simulink model "SMXQ6_600_GoKart_Project"  (R2026a)
settings: Solver=VariableStepAuto  StopTime=7
model workspace (MAT data in the model file):
  CruiseSpeed = 1
  DaxisKi = 3000
  DaxisKp = 18
  InvThresh = 1
  MaxPower = 2638
  MaxTorque = 42
  NPP = 20
  QaxisKi = 3000
  QaxisKp = 18
  SpeedKi = 2882.18001217
  SpeedKp = 90.4773949421
  Tf = 0.0001
  Ts = 0.0001
  Vdc = 320
  flux = 0.103309826163
  speedramp = [0 0.125 0.125 0.5 0.5 1 1]
  timeramp = [0 1 2 3 4 5 6]
libraries: fl_lib x15, nesl_utility x15, sdl_lib x6, ee_lib x4, slpidlib x1, eePmsmFieldOrientedControl x1
(part 1 of 2)
settings Model: Creator=bneiswan  LastModifiedBy=Uriel
settings SimscapeCC: SimscapeNominalValues="[{\"value\":\"1\",\"unit\":\"A\"},{\"value\":\"1\",\"unit\":\"bar\"},{\"value\":\"1\",\"unit\":\"cm^2\"},{\"value\":\"1\",\"unit\":\"cm^3/s\"},{\"value\":\"1\",\"unit\":\"kJ/kg\"},{\"value\":\"1\",\"unit\":\"kW\"},{\"value\":\"1\",\"unit\":\"l\"},{\"value\":\"1\",\"unit\":\"N\"},{\"value\":\"1\",\"unit\":\"N*m\"},{\"value\":\"1\",\"unit\":\"V\"}]"  SimscapeLogType=none  SimscapeLogDataHistory=5000.0

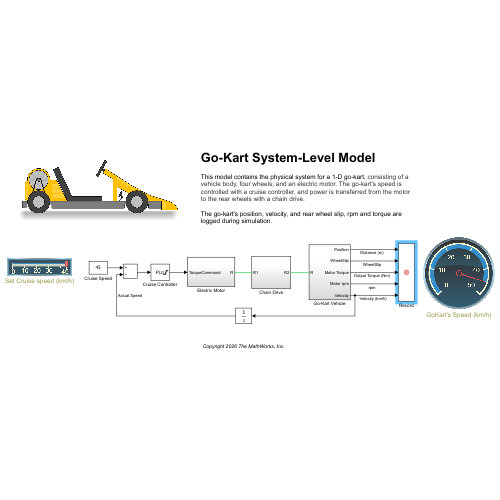
[thumbnail: Simulink's stored preview of the top-level diagram]
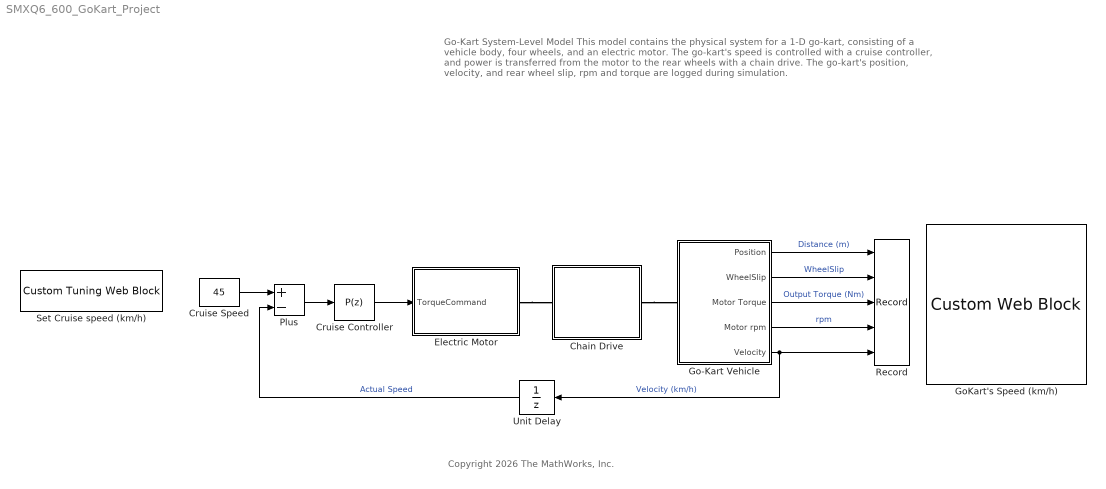
== system SMXQ6_600_GoKart_Project ==
  note: Copyright 2026 The MathWorks, Inc.
  note: Go-Kart System-Level Model
      |
      | This model contains the physical system for a 1-D go-kart, consisting of a vehicle body, four wheels, and an electric motor. The go-kart's speed is controlled with a cruise controller, and power is transferred from the motor to the rear wheels with a chain drive.
      |
      | The go-kart's position, velocity, and rear wheel slip, rpm and torque are logged during simulation.
  Chain Drive : Subsystem
  Cruise Controller : slpidlib/PID Controller  Controller=P  Form=Parallel  TimeDomain=Discrete-time  UseExternalTs=off  SampleTime=-1  IntegratorMethod=Forward Euler  FilterMethod=Forward Euler  ControllerParametersSource=internal  P=250  I=.25  UseKiTs=off  D=10  UseExternalDerivativeSource=off  N=100  UseFilter=on  TunerSelectOption=Transfer Function Based (PID Tuner App)  InitialConditionSource=internal  InitialConditionForIntegrator=0  InitialConditionForFilter=0  DifferentiatorICPrevScaledInput=0  ExternalReset=none  TrackingMode=off  Kt=1  LimitOutput=on  SatLimitsSource=internal  UpperSaturationLimit=42  LowerSaturationLimit=0  LinearizeAsGain=on  AntiWindupMode=none  Kb=1  LimitIntegrator=off  UpperIntegratorSaturationLimit=inf  LowerIntegratorSaturationLimit=-inf  POutMin=[]  POutMax=[]  IOutMin=[]  IOutMax=[]  DOutMin=[]  DOutMax=[]  NOutMin=[]  NOutMax=[]  SumOutMin=[]  SumOutMax=[]  SaturationOutMin=[]  SaturationOutMax=[]  PParamMin=[]  PParamMax=[]  IParamMin=[]  IParamMax=[]  DParamMin=[]  DParamMax=[]  NParamMin=[]  NParamMax=[]  KbParamMin=[]  KbParamMax=[]  KtParamMin=[]  KtParamMax=[]  KbOutMin=[]  KbOutMax=[]  KtOutMin=[]  KtOutMax=[]  IntegratorOutMin=[]  IntegratorOutMax=[]  FilterOutMin=[]  FilterOutMax=[]  SumI1OutMin=[]  SumI1OutMax=[]  SumI2OutMin=[]  SumI2OutMax=[]  SumI3OutMin=[]  SumI3OutMax=[]  SumI4OutMin=[]  SumI4OutMax=[]  SumDOutMin=[]  SumDOutMax=[]  DifferentiatorOutMin=[]  DifferentiatorOutMax=[]  FilterDiffOutCoefMin=[]  FilterDiffOutCoefMax=[]  ReciprocalOutMin=[]  ReciprocalOutMax=[]  SumDenOutMin=[]  SumDenOutMax=[]  SumNumOutMin=[]  SumNumOutMax=[]  DivideOutMin=[]  DivideOutMax=[]  UdiffTsProdOutMin=[]  UdiffTsProdOutMax=[]  NTsProdOutMin=[]  NTsProdOutMax=[]  UintegralTsProdOutMin=[]  UintegralTsProdOutMax=[]  UngainTsProdOutMin=[]  UngainTsProdOutMax=[]  ClampingZeroOutDataTypeStr=Inherit: Inherit via back propagation  ClampingZeroOutMin=[]  ClampingZeroOutMax=[]  FilterDenConstantOutDataTypeStr=Inherit: Inherit via back propagation  FilterDenConstantOutMin=[]  FilterDenConstantOutMax=[]  PCopyOutDataTypeStr=Inherit: Inherit via back propagation  PCopyOutMin=[]  PCopyOutMax=[]  NCopyOutDataTypeStr=Inherit: Inherit via back propagation  NCopyOutMin=[]  NCopyOutMax=[]  IntegratorContinuousStateAttributes=''  IntegratorStateMustResolveToSignalObject=off  IntegratorRTWStateStorageClass=Auto  FilterContinuousStateAttributes=''  FilterStateMustResolveToSignalObject=off  FilterRTWStateStorageClass=Auto  ParallelPVariant=InternalParameters  IdealPVariant=Disabled  IVariant=Disabled  DVariant=Disabled  IntegratorVariant=Disabled  SatVariant=Enabled  AWVariant=Disabled  PCopyVariant=Disabled  TRVariant=Disabled  FdbkBlocksVariant=Forward  IdealPFdbkVariant=Disabled  SatFdbkVariant=Disabled  DerivativeFilterVariant=Disabled  NVariant=Disabled  NCopyVariant=Disabled_SignalSpec  FilterICVariant=Disabled  IntegratorICVariant=Disabled  ExternalResetVariant=Disabled  TRSumVariant=Passthrough  SumFdbkVariant=Disabled  SumVariant=Passthrough_P  TsampFilterVariant=InternalTs  TsampNgainVariant=Passthrough  TsampIntegralVariant=Disabled_SignalSpec  ExternalSaturationOutDataTypeStr=Inherit: Same as second input  DerivativeSourceVariant=Disabled  PreIntVariant=InternalPreInt
  Cruise Speed : Constant  Value=45
  Electric Motor : Subsystem
      settings: PortSchema="{\"entries\":[{\"content\":{\"sides\":[{\"content\":{\"connectorIds\":[\"LConn1\"]},\"type\":\"ConnectorPlacement.EquallySpacedRectSide\",\"uuid\":\"f2a7d976-2b6b-46c6-a0c1-1e92cd96bdba\"},{\"content\":{\"connectorIds\":[\"In1\"],\"side\":\"RIGHT\"},\"type\":\"ConnectorPlacement.EquallySpacedRectSide\",\"uuid\":\"0fb82cfe-b0ae-4149-8652-d7e7f0635458\"},{\"content\":{\"side\":\"TOP\"},\"type\":\"ConnectorPlacement.EquallySpacedRectSide\",\"uuid\":\"f6564529-e6f3-4994-b1c4-046997b74a0b\"}]},\"type\":\"ConnectorPlacement.EquallySpacedConnector\",\"uuid\":\"916fedef-c12c-4718-8891-25d762e09ffe\"}],\"packageUris\":[\"http://schema.mathworks.com/mf0/Connector/R2020b\"],\"version\":\"1.0\"}"
  Go-Kart Vehicle : Subsystem
  GoKart's Speed (km/h) : CustomWebBlock  LabelPosition=Hide  ShowInitialText=on  Configuration="{\"components\":[{\"name\":\"CircularScaleComponent\",\"settings\":{\"bounds\":{\"max\":50,\"min\":0,\"tickInterval\":5},\"direction\":\"cw\",\"flipLimits\":0,\"innerRadius\":0.75,\"internalTickHeightScaleFactor\":1,\"labelColor\":[255,255,200],\"labelFont\":{\"font\":\"Arial\",\"fontSize\":12},\"labelRadius\":0.528,\"labelTransparency\":1,\"minorTickHeightScaleFactor\":0.2,\"needleImage\":{\"size\":[200,50],\"src\":\"data:image\\/svg+xml;base64,PD94bWwgdmVyc2lvbj0iMS4wIiBlbmNvZGluZz0idXRmLTgiPz4KPCEtLSBHZW5lcmF0b3I6IEFkb2JlIElsbHVzdHJhdG9yIDI0LjEuMiwgU1ZHIEV4cG9ydCBQbHVnLUluIC4gU1ZHIFZlcnNpb246IDYuMDAgQnVpbGQgMCkgIC0tPgo8c3ZnIHZlcnNpb249IjEuMSIgaWQ9IkxheWVyXzEiIHhtbG5zPSJodHRwOi8vd3d3LnczLm9yZy8yMDAwL3N2ZyIgeG1sbnM6eGxpbms9Imh0dHA6Ly93d3cudzMub3JnLzE5OTkveGxpbmsiIHg9IjBweCIgeT0iMHB4IgoJIHZpZXdCb3g9IjAgMCAyMDAgNTAiIHN0eWxlPSJlbmFibGUtYmFja2dyb3VuZDpuZXcgMCAwIDIwMCA1MDsiIHhtbDpzcGFjZT0icHJlc2VydmUiPgo8c3R5bGUgdHlwZT0idGV4dC9jc3MiPgoJLnN0MHtmaWxsOiNFQzIxMjc7fQo8L3N0eWxlPgo8cGF0aCBjbGFzcz0ic3QwIiBkPSJNMTYyLjgsMTMuN0MxNjksNC40LDE4MS43LDEuOSwxOTEsOC4xczExLjgsMTguOSw1LjYsMjguMnMtMTguOSwxMS44LTI4LjIsNS42bDAsMAoJQzE1OS4xLDM1LjYsMTU2LjYsMjMsMTYyLjgsMTMuN0wxNjIuOCwxMy43eiBNMTY1LjgsMTUuOGMtNS4xLDcuNi0zLjEsMTcuOSw0LjYsMjNjNy42LDUuMSwxNy45LDMuMSwyMy00LjYKCWM1LjEtNy42LDMuMS0xNy45LTQuNi0yM2wwLDBDMTgxLjIsNi4yLDE3MC45LDguMiwxNjUuOCwxNS44eiIvPgo8cGF0aCBjbGFzcz0ic3QwIiBkPSJNMC40LDI1Ljl2LTMuM2wxNTktMi41Yy0wLjcsMi42LTAuNyw1LjIsMCw3LjhMMC40LDI1Ljl6Ii8+CjxjaXJjbGUgY2xhc3M9InN0MCIgY3g9IjE3OS42IiBjeT0iMjQiIHI9IjAuNyIvPgo8L3N2Zz4K\"},\"needleOffset\":[0.18464878250906522,0],\"needleOrientation\":-45,\"needleRotation\":180,\"needleSize\":{\"height\":0.11741692305346914,\"width\":0.46108337545091255},\"outerRadius\":0.9,\"position\":[0.05,0.05,0.9,0.9],\"referencePoint\":\"auto\",\"scaleAngle\":270,\"scaleAngleOffset\":135,\"scaleColors\":[],\"scaleColorsSize\":0.2,\"scaleDirection\":\"CW\",\"scalePosition\":[0,0,1,1],\"showLabels\":1,\"showMinorTicks\":1,\"showSpanLine\":1,\"showTicks\":1,\"tickColor\":[252,252,197],\"tickTransparency\":1,\"valueBarColor\":[0,114,189],\"valueBarPosition\":[0,0,1,1],\"valueBarSize\":0.2,\"valueBarTransparency\":1}},{\"name\":\"BackgroundImageComponent\",\"settings\":{\"image\":{\"size\":[500,500],\"src\":\"data:image\\/svg+xml;base64,PD94bWwgdmVyc2lvbj0iMS4wIiBlbmNvZGluZz0iVVRGLTgiIHN0YW5kYWxvbmU9Im5vIj8+CjxzdmcKICAgeG1sbnM6ZGM9Imh0dHA6Ly9wdXJsLm9yZy9kYy9lbGVtZW50cy8xLjEvIgogICB4bWxuczpjYz0iaHR0cDovL2NyZWF0aXZlY29tbW9ucy5vcmcvbnMjIgogICB4bWxuczpyZGY9Imh0dHA6Ly93d3cudzMub3JnLzE5OTkvMDIvMjItcmRmLXN5bnRheC1ucyMiCiAgIHhtbG5zOnN2Zz0iaHR0cDovL3d3dy53My5vcmcvMjAwMC9zdmciCiAgIHhtbG5zPSJodHRwOi8vd3d3LnczLm9yZy8yMDAwL3N2ZyIKICAgeG1sbnM6 ...(+9964 chars)\"},\"position\":[0,0,1,1],\"scaleMode\":\"0\"}},{\"name\":\"ForegroundImageComponent\",\"settings\":{\"image\":{\"size\":[0,0],\"src\":\"default\",\"srcOrientation\":[]},\"isForeground\":1,\"position\":[0,0,1,1],\"scaleMode\":\"0\"}}],\"derived\":{\"blockParameters\":{\"ForegroundColor\":[0.9882352941176471,0.9882352941176471,0.7725490196078432],\"Limits\":{\"Max\":50,\"Min\":0,\"Ticks\":5},\"ScaleColors\":[],\"ScaleDirection\":\"Clockwise\",\"ScaleMax\":50,\"ScaleMin\":0,\"TickInterval\":5,\"fixedAspectRatio\":\"on\"}},\"settings\":{\"BindingType\":\"signal\",\"aspectRatio\":1.032258064516129,\"backgroundColor\":[0,0,0,\"1\"],\"backgroundOffset\":1,\"backgroundOpacity\":1,\"direction\":\"cw\",\"fixedAspectRatio\":\"on\",\"flipLimits\":0,\"orientation\":\"horizontal\",\"showBackgroundColor\":false,\"value\":0,\"version\":\"R2023a\"},\"type\":\"CircularGauge\"}"
  Plus : Sum  Inputs=+-
  Record : Record  NumPorts=5.0  FileSettingsInternal="{\"entries\":[{\"content\":{\"excelSettings\":{\"content\":{},\"type\":\"Streamout.ExcelSettings\"},\"parquetSettings\":{\"content\":{},\"type\":\"Streamout.ParquetSettings\"}},\"type\":\"Streamout.FileSettingStorage\",\"uuid\":\"\"}],\"packageUris\":[\"http:\\/\\/schema.mathworks.com\\/mf0\\/streamout_blocks\\/R2020a\"],\"version\":\"1.0\"}"  FrameSettings=[0, 0, 0, 0, 0]  SignalsInternal="{\"entries\":[{\"content\":{\"signals\":[{\"content\":{\"blockPath\":[],\"dimensions\":[1],\"domain\":\"\",\"lineColor\":\"#0072bd\",\"lineWidth\":2,\"plots\":[ 1 ],\"port\":1,\"sid\":[\"\"],\"signalID\":1,\"signalName\":\"Distance (m)\"},\"type\":\"RecordBlkView.Signal\",\"uuid\":\"\"},{\"content\":{\"blockPath\":[],\"dimensions\":[1],\"domain\":\"\",\"lineColor\":\"#d95319\",\"lineWidth\":2,\"plots\":[ 1 ],\"port\":2,\"sid\":[\"\"],\"signalID\":2,\"signalName\":\"WheelSlip\"},\"type\":\"RecordBlkView.Signal\",\"uuid\":\"\"},{\"content\":{\"blockPath\":[],\"dimensions\":[1],\"domain\":\"\",\"lineColor\":\"#edb120\",\"lineWidth\":2,\"plots\":[ 1 ],\"port\":3,\"sid\":[\"\"],\"signalID\":3,\"signalName\":\"Output Torque (Nm)\"},\"type\":\"RecordBlkView.Signal\",\"uuid\":\"\"},{\"content\":{\"blockPath\":[],\"dimensions\":[1],\"domain\":\"\",\"lineColor\":\"#7e2f8e\",\"lineWidth\":2,\"plots\":[ 1 ],\"port\":4,\"sid\":[\"\"],\"signalID\":4,\"signalName\":\"rpm\"},\"type\":\"RecordBlkView.Signal\",\"uuid\":\"\"},{\"content\":{\"blockPath\":[],\"dimensions\":[1],\"domain\":\"\",\"lineColor\":\"#77ac30\",\"lineWidth\":2,\"plots\":[ 1 ],\"port\":5,\"sid\":[\"\"],\"signalID\":5,\"signalName\":\"Velocity (km\\/h)\"},\"type\":\"RecordBlkView.Signal\",\"uuid\":\"\"}]},\"type\":\"RecordBlkView.InputSignals\",\"uuid\":\"\"}],\"packageUris\":[\"http:\\/\\/schema.mathworks.com\\/mf0\\/streamout_blocks\\/R2020a\"],\"version\":\"1.0\"}"  VisualizationBindings="{\"sparklinesplugin\":{\"info\":[{\"bindingParametersList\":[],\"subplotID\":1}]}}"
  Set Cruise speed (km/h) : CustomTuningWebBlock  LabelPosition=Hide  ShowInitialText=on  Configuration="{\"components\":[{\"name\":\"LinearScaleComponent\",\"settings\":{\"bounds\":{\"max\":45,\"min\":0,\"tickInterval\":\"auto\"},\"internalTickHeightScaleFactor\":0.5,\"labelColor\":[255,255,200],\"labelFont\":{\"font\":\"Arial\",\"fontSize\":12},\"labelOffset\":0.05,\"labelTransparency\":1,\"needleImage\":{\"size\":[596,842],\"src\":\"data:image\\/svg+xml;base64,PD94bWwgdmVyc2lvbj0iMS4wIiBlbmNvZGluZz0idXRmLTgiPz4NCjwhLS0gR2VuZXJhdG9yOiBBZG9iZSBJbGx1c3RyYXRvciAyNS4wLjAsIFNWRyBFeHBvcnQgUGx1Zy1JbiAuIFNWRyBWZXJzaW9uOiA2LjAwIEJ1aWxkIDApICAtLT4NCjxzdmcgdmVyc2lvbj0iMS4xIg0KCSBpZD0ic3ZnOCIgeG1sbnM6Y2M9Imh0dHA6Ly9jcmVhdGl2ZWNvbW1vbnMub3JnL25zIyIgeG1sbnM6ZGM9Imh0dHA6Ly9wdXJsLm9yZy9kYy9lbGVtZW50cy8xLjEvIiB4bWxuczppbmtzY2FwZT0iaHR0cDovL3d3dy5pbmtzY2FwZS5vcmcvbmFtZXNw ...(+2420 chars)\",\"srcOrientation\":\"Right\"},\"needleOffset\":[-0.8044596912521441,-0.0642123287671233],\"needleSize\":{\"height\":0.4337797619047619,\"width\":0.07668067226890757},\"position\":[0.2829861111111111,0.04398634453781513,0.9196428571428571,0.6088789682539683],\"referencePoint\":\"auto\",\"scaleColors\":[],\"scaleColorsSize\":0.2,\"scaleDirection\":\"LR\",\"showLabels\":1,\"showMinorTicks\":0,\"showSpanLine\":1,\"showTicks\":1,\"tickColor\":[252,252,197],\"tickTransparency\":1,\"valueBarColor\":[0,114,189],\"valueBarOffset\":-0.27,\"valueBarSize\":0.1,\"valueBarTransparency\":1}},{\"name\":\"BackgroundImageComponent\",\"settings\":{\"image\":{\"size\":[380,101],\"src\":\"data:image\\/svg+xml;base64,PHN2ZyB4bWxucz0iaHR0cDovL3d3dy53My5vcmcvMjAwMC9zdmciIHhtbG5zOnhsaW5rPSJodHRwOi8vd3d3LnczLm9yZy8xOTk5L3hsaW5rIiB2aWV3Qm94PSIwIDAgMzgwIDEwMSI+PGRlZnM+PHN0eWxlPi5jbHMtMXtmaWxsOiMwMDJiNDI7fS5jbHMtMntmaWxsOiM0MjcwODI7fS5jbHMtM3tmaWxsOnVybCgjcmFkaWFsLWdyYWRpZW50KTt9LmNscy00e2ZpbGw6I2M4YzhjODtzdHJva2U6IzAwMDt9PC9zdHlsZT48cmFkaWFsR3JhZGllbnQgaWQ9InJhZGlhbC1ncmFkaWVudCIgY3g9IjE5MCIgY3k9IjUwLjUiIHI9IjI2OS4yMSIgZ3JhZGllbnRVbml0cz0idXNlclNwYWNlT25Vc2UiPjxzdG9wIG9mZnNldD0iMC4wMSIgc3RvcC1jb2xvcj0iIzNlNGY1OCIvPjxzdG9wIG9mZnNldD0iMC4wNiIgc3RvcC1jb2xvcj0iIzQ0NTc2MSIvPjxzdG9wIG9mZnNldD0iMC4xNSIgc3RvcC1jb2xvcj0iIzU1NmE3NiIvPjxzdG9wIG9mZnNldD0iMC4yNSIgc3RvcC1jb2xvcj0iIzZkODg5NSIvPjxzdG9wIG9mZnNldD0iMC4zOCIgc3RvcC1jb2xvcj0iIzhmYjJjMyIvPjxzdG9wIG9mZnNldD0iMC41MiIgc3RvcC1jb2xvcj0iI2I2ZTRmYSIvPjxzdG9wIG9mZnNldD0iMSIgc3RvcC1jb2xvcj0iIzE1NDY1NyIvPjwvcmFkaWFsR3JhZGllbnQ+PC9kZWZzPjxnIGlkPSJmcmFtZSI+PGcgaWQ9IkxheWVyXzIiIGRhdGEtbmFtZT0iTGF5ZXIgMiI+PGcgaWQ9IkxheWVyXzEtMiIgZGF0YS1uYW1lPSJMYXllciAxLTIiPjxyZWN0IGlkPSJyZWN0MTAzNiIgY2xhc3M9ImNscy0xIiB4PSIxMSIgeT0iMTEiIHdpZHRoPSIzNTgiIGhlaWdodD0iNzkiLz48cGF0aCBpZD0icGF0aDEwMzgiIGNsYXNzPSJjbHMtMiIgZD0iTTgsOFY5M0gzNzJWOFpNMzY5LDkwSDExVjExSDM2OVoiLz48cGF0aCBpZD0icGF0aDEwNDAiIGNsYXNzPSJjbHMtMyIgZD0iTTAsMFYxMDFIMzgwVjBaTTM3Miw5M0g4VjhIMzcyWiIvPjwvZz48L2c+PC9nPjxnIGlkPSJ0cmFjayI+PHBhdGggaWQ9InJlY3QxNjExIiBjbGFzcz0iY2xzLTQiIGQ9Ik0zMy4zNywyNi41OUgzNDYuNjNjNCwwLDcuMjUsMi42LDcuMjUsNS44MWgwYzAsMy4yMS0zLjI1LDUuODItNy4yNSw1LjgySDMzLjM3Yy00LDAtNy4yNS0yLjYxLTcuMjUtNS44MmgwQzI2LjEyLDI5LjE5LDI5LjM3LDI2LjU5LDMzLjM3LDI2LjU5WiIvPjwvZz48L3N2Zz4=\",\"srcOrientation\":\"horizontal\"},\"position\":[0,0,1,1],\"scaleMode\":\"0\"}},{\"name\":\"ForegroundImageComponent\",\"settings\":{\"image\":{\"size\":[0,0],\"src\":\"default\",\"srcOrientation\":[]},\"isForeground\":1,\"position\":[0,0,1,1],\"scaleMode\":\"0\"}}],\"derived\":{\"blockParameters\":{\"ForegroundColor\":[0.9882352941176471,0.9882352941176471,0.7725490196078432],\"Limits\":{\"Max\":45,\"Min\":0,\"Ticks\":\"auto\"},\"ScaleColors\":[],\"ScaleDirection\":\"Clockwise\",\"ScaleMax\":45,\"ScaleMin\":0,\"TickInterval\":\"auto\",\"fixedAspectRatio\":\"on\"}},\"settings\":{\"BindingType\":\"param\",\"aspectRatio\":3.7777777777777777,\"backgroundColor\":[0,0,0,\"1\"],\"backgroundOffset\":0,\"backgroundOpacity\":1,\"fixedAspectRatio\":\"on\",\"foregroundColor\":[252,252,196],\"orientation\":\"horizontal\",\"showBackgroundColor\":false,\"value\":0,\"version\":\"R2023a\"},\"type\":\"LinearGauge\"}"
  Unit Delay : UnitDelay  SampleTime=-1
  wires:
  Cruise Speed/1 -> Plus/1
  Plus/1 -> Cruise Controller/1
  Cruise Controller/1 -> Electric Motor/1(TorqueCommand)
  Unit Delay/1 -> Plus/2  "Actual Speed"
  Go-Kart Vehicle/4(Motor rpm) -> Record/4  "rpm"
  Go-Kart Vehicle/1(Position) -> Record/1  "Distance (m)"
  Go-Kart Vehicle/3(Motor Torque) -> Record/3  "Output Torque (Nm)"
  Go-Kart Vehicle/5(Velocity) -> Unit Delay/1, Record/5  "Velocity (km/h)"
  Go-Kart Vehicle/2(WheelSlip) -> Record/2  "WheelSlip"
  connections:
  Chain Drive/RConn1 -- Go-Kart Vehicle/LConn1
  Electric Motor/LConn1 -- Chain Drive/LConn1

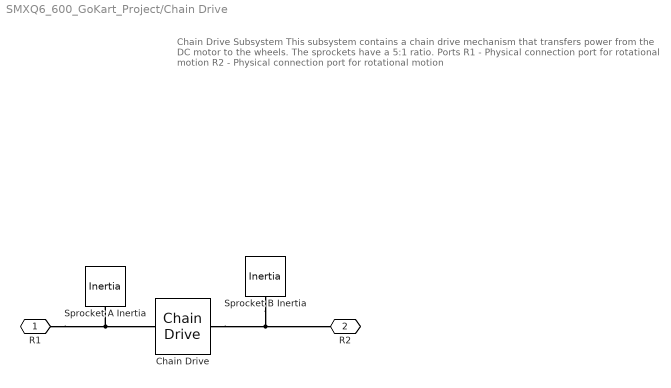
== system SMXQ6_600_GoKart_Project/Chain Drive ==
  note: Chain Drive Subsystem
      |
      | This subsystem contains a chain drive mechanism that transfers power from the DC motor to the wheels. The sprockets have a 5:1 ratio.
      |
      | Ports
      | R1 - Physical connection port for rotational motion
      | R2 - Physical connection port for rotational motion
  Chain Drive : sdl_lib/Couplings & Drives/Chain Drive  chain_model=sdl.enum.chain_model.ideal  radius_a=2 cm  radius_b=3 cm  slack=50 mm  k_chain=1e5 N/m  mu_visc_chain=5 N*s/m  mu_visc_a=0.001 N*m*s/rad  mu_visc_b=0.001 N*m*s/rad  breakable=sdl.enum.max_tension.off  F_max=1e6 N  x_specify=off  x_priority=High  x=0 mm  x_nominal_specify=off  x_nominal_value=1  x_nominal_unit=mm
  Sprocket A Inertia : fl_lib/Mechanical/Rotational Elements/Inertia  inertia=0.002 kg*m^2  num_ports=foundation.enum.numPorts2.one  w_specify=off  w_priority=High  w=0 rad/s  w_nominal_specify=off  w_nominal_value=1  w_nominal_unit=rad/s  t_specify=off  t_priority=None  t=0 N*m  t_nominal_specify=off  t_nominal_value=1  t_nominal_unit=N*m
  Sprocket B Inertia : fl_lib/Mechanical/Rotational Elements/Inertia  inertia=0.2 kg*m^2  num_ports=foundation.enum.numPorts2.one  w_specify=off  w_priority=High  w=0 rad/s  w_nominal_specify=off  w_nominal_value=1  w_nominal_unit=rad/s  t_specify=off  t_priority=None  t=0 N*m  t_nominal_specify=off  t_nominal_value=1  t_nominal_unit=N*m
  R1 : PMIOPort  Side=Left
  R2 : PMIOPort  Port=2  Side=Right
  connections:
  Sprocket B Inertia/LConn1 -- R2/RConn1 -- Chain Drive/RConn1
  R1/RConn1 -- Chain Drive/LConn1 -- Sprocket A Inertia/LConn1

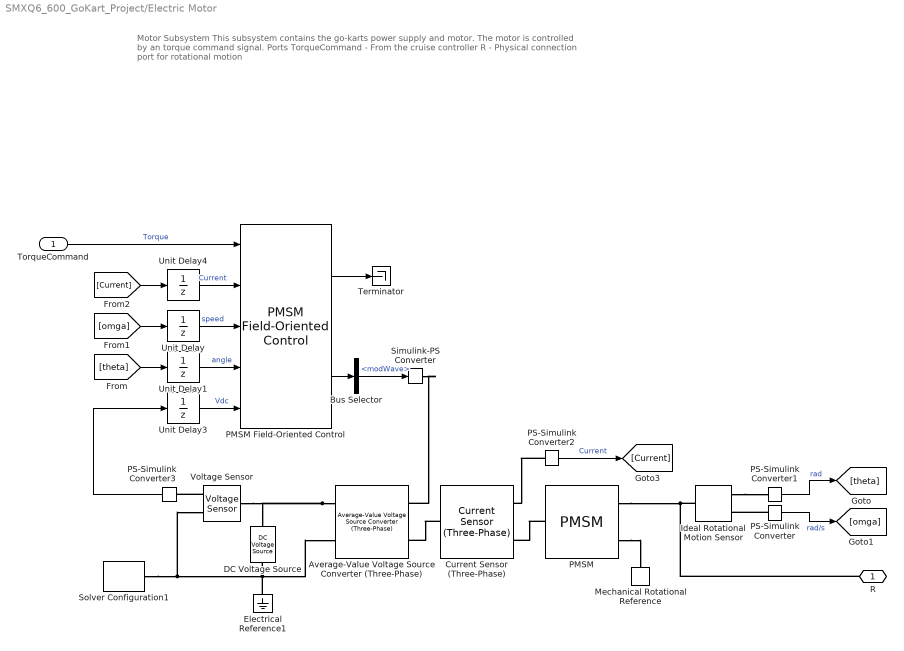
== system SMXQ6_600_GoKart_Project/Electric Motor ==
  note: Motor Subsystem
      |
      | This subsystem contains the go-karts power supply and motor. The motor is controlled by an torque command signal.
      |
      | Ports
      | TorqueCommand - From the cruise controller
      | R - Physical connection port for rotational motion
  TorqueCommand : Inport
  Average-Value Voltage Source Converter (Three-Phase) : ee_lib/Semiconductors & Converters/Converters/Average-Value Voltage Source Converter (Three-Phase)  port_option=ee.enum.threePhasePort.composite  enable_block_pulses_input=false  krec=0.01 Ohm  frequency_option=ee.enum.converters.frequency.variable  input_option=ee.enum.converters.inputOption.ModWave  FRated=60 Hz  losses_parameterization=ee.enum.converters.losses.fixed  Pfixed=1 W  ks=0.01  kc1=1.7 V  kc2=0.01 Ohm  Ploss_vect=[100, 800, 1870, 3250, 4900] W  Irms_vect=[10, 100, 200, 300, 400] A  Vdc_nom=300 V  thermal_mass=30000 J/K  temperature_specify=off  temperature_priority=High  temperature=298.15 K  temperature_nominal_specify=off  temperature_nominal_value=1  temperature_nominal_unit=K
  Bus Selector : BusSelector  OutputSignals=modWave
  Current Sensor (Three-Phase) : ee_lib/Sensors & Transducers/Current Sensor (Three-Phase)  port_option=ee.enum.threePhasePort.composite
  DC Voltage Source : ee_lib/Additional Components/SPICE Sources/DC Voltage Source  DC=320 V
      settings: AttributesFormatString=%<DC>%<DC_unit>
  Electrical Reference1 : fl_lib/Electrical/Electrical Elements/Electrical Reference
  Ideal Rotational Motion Sensor : fl_lib/Mechanical/Mechanical Sensors/Ideal Rotational Motion Sensor  reference=foundation.enum.MeasurementReference.absolute  acceleration_port=false  velocity_port=true  position_port=true  wrap_angle=false  offset=0 rad
  Mechanical Rotational Reference : fl_lib/Mechanical/Rotational Elements/Mechanical Rotational Reference
  PMSM : ee_lib/Electromechanical/Permanent Magnet/PMSM  PartSpecification="{\"CollectionId\":\"MW.SimscapeElectrical\",\"CollectionVersion\":\"1.0.0\",\"DatasetId\":\"Swiss_Mekatronix|SMXQ6-600|simscape.electrical.pmsm\",\"DisplayName\":\"Swiss_Mekatronix:SMXQ6-600\"}"  port_option=ee.enum.threePhasePort.composite  winding_type=ee.enum.electromech.statorconfiguration.wye  machine_param=ee.enum.pmsm.parameterization.constant  nPolePairs=20 % Datasheet derived  pmflux_param=ee.enum.pmflux.fluxlinkage  pm_flux_linkage=0.103309826163462 % Datasheet derived Wb  torque_constant=2.06619652326924 % Datasheet derived N*m/A  back_emf_constant=2.06619652326924 % Datasheet derived V/(rad/s)  stator_param=ee.enum.statorparam.LdLqL0  Ld=0.0018 % Datasheet derived H  Lq=0.0018 % Datasheet derived H  idVec=[-200, 0, 200] % Parameter not set A  iqVec=[-200, 0, 200] % Parameter not set A  LdMatrix=0.0002 * ones(3, 3) % Parameter not set H  LqMatrix=0.0002 * ones(3, 3) % Parameter not set H  PmMatrix=0.1 * ones(3, 3) % Parameter not set Wb  ktMatrix=[0.18 0.18 0.18;0.18 0.18 0.18;0.18 0.18 0.18] % Datasheet derived N*m/A  keMatrix=0.18 * ones(3, 3) % Parameter not set V*s/rad  L0=0.00016 % Parameter not set H  Ls=0.0002 % Parameter not set H  Lm=-0.00002 % Parameter not set H  Ms=0.00002 % Parameter not set H  Rs=0.3 % Datasheet derived Ohm  zero_sequence=ee.enum.park.zerosequence.exclude  axes_param=ee.enum.rotorangle.daxis  loss_param=ee.enum.ironloss.none  losses_oc=[0, 0, 0] % Parameter not set W  losses_sc=[0, 0, 0] % Parameter not set W  f_losses=60 % Parameter not set Hz  Isc_losses=95 % Parameter not set A  J=0.0243 % Datasheet derived kg*m^2  lam=0 % Parameter not set N*m*s/rad  i_d_specify=off  i_d_priority=None  i_d=0 A  i_d_nominal_specify=off  i_d_nominal_value=1  i_d_nominal_unit=A  i_q_specify=off  i_q_priority=None  i_q=0 A  i_q_nominal_specify=off  i_q_nominal_value=1  i_q_nominal_unit=A  torque_specify=off  torque_priority=None  torque=0 N*m  torque_nominal_specify=off  torque_nominal_value=1  torque_nominal_unit=N*m  angular_velocity_specify=off  angular_velocity_priority=High  angular_velocity=0 rpm  angular_velocity_nominal_specify=off  angular_velocity_nominal_value=1  angular_velocity_nominal_unit=rpm  angular_position_specify=off  angular_position_priority=High  angular_position=0 deg  angular_position_nominal_specify=off  angular_position_nominal_value=1  angular_position_nominal_unit=deg  alpha=3.93e-3 % Parameter not set 1/K  alpha_flux=-0.001 % Parameter not set 1/K  Tmeas=298.15 % Parameter not set K  stator_thermal_mass=100 % Parameter not set J/K  rotor_thermal_mass=200 % Parameter not set J/K  Rm_percent_rotor=90 % Parameter not set  Rd_percent_rotor=30 % Parameter not set  temperatureA_specify=off  temperatureA_priority=High  temperatureA=25 degC  temperatureA_nominal_specify=off  temperatureA_nominal_value=1  temperatureA_nominal_unit=degC  temperatureB_specify=off  temperatureB_priority=High  temperatureB=25 degC  temperatureB_nominal_specify=off  temperatureB_nominal_value=1  temperatureB_nominal_unit=degC  temperatureC_specify=off  temperatureC_priority=High  temperatureC=25 degC  temperatureC_nominal_specify=off  temperatureC_nominal_value=1  temperatureC_nominal_unit=degC  temperatureR_specify=off  temperatureR_priority=High  temperatureR=25 degC  temperatureR_nominal_specify=off  temperatureR_nominal_value=1  temperatureR_nominal_unit=degC
      settings: AttributesFormatString=Swiss_Mekatronix:SMXQ6-600
  PMSM Field-Oriented Control : eePmsmFieldOrientedControl/PMSM Field-Oriented Control  winding_type=Wye-wound  CtrlMode=Torque control  Vnom=Vdc  Pmax=MaxPower  Tmax=MaxTorque  p=NPP  Vdc_on=InvThresh  Ts=Tf  Tsc=Ts  CtrlType=PI control  Kp_w=0  Ki_w=0  Kv_w=1  Kaw_w=0  RefType=Zero d-axis control  rpmVec=[0, 3000]  TqVec=[-100, 0, 100]  VdcVec=[300, 350]  PWMMode=SPWM: sinusoidal PWM  ModFactor=1  idMatrix=zeros(2,3,2)  iqMatrix=zeros(2,3,2)  psim=flux  Ld=0.00024  Lq=0.00029  Rs=0.01  AxisAlignment=D-axis  Kp_id=DaxisKp  Ki_id=DaxisKi  Kaw_id=1  Kp_iq=QaxisKp  Ki_iq=QaxisKi  Kaw_iq=1  AxisPrio=Q-axis  ActZC=off  ActFF=off  ParamTypeFF=Constant parameters  LdFF=0  LqFF=0  psimFF=0  idVect=[-200, 0, 200]  iqVect=[-200, 0, 200]  LdMatrix=0.0002 * ones(3, 3)  LqMatrix=0.0002 * ones(3, 3)  psimMatrix=0.04 * ones(3, 3)  CPWMMode=SPWM: sinusoidal PWM  fsw=1000
      settings: LibrarySourceBlock=|
      | ee_sl_lib/PMSM Control/PMSM Field-Oriented
      | Control
  PS-Simulink Converter : nesl_utility/PS-Simulink Converter  PhysicalDomain=network_engine_domain  SubClassName=ps_output  LeftPortType=input  RightPortType=output  PseudoPeriodic=off  Frequencies=[]  VectorFormat=inherit  Unit=rad/s  AffineConversion=off
  PS-Simulink Converter1 : nesl_utility/PS-Simulink Converter  PhysicalDomain=network_engine_domain  SubClassName=ps_output  LeftPortType=input  RightPortType=output  PseudoPeriodic=off  Frequencies=[]  VectorFormat=inherit  Unit=rad  AffineConversion=off
  PS-Simulink Converter2 : nesl_utility/PS-Simulink Converter  PhysicalDomain=network_engine_domain  SubClassName=ps_output  LeftPortType=input  RightPortType=output  PseudoPeriodic=off  Frequencies=[]  VectorFormat=inherit  Unit=inherit  AffineConversion=off
  PS-Simulink Converter3 : nesl_utility/PS-Simulink Converter  PhysicalDomain=network_engine_domain  SubClassName=ps_output  LeftPortType=input  RightPortType=output  PseudoPeriodic=off  Frequencies=[]  VectorFormat=inherit  Unit=inherit  AffineConversion=off
  Simulink-PS Converter : nesl_utility/Simulink-PS Converter  PhysicalDomain=network_engine_domain  SubClassName=ps_input  LeftPortType=input  RightPortType=output  PseudoPeriodic=off  Frequencies=[]  NoiseDistribution=none  NoiseParameters=[]  Unit=1  AffineConversion=off  FilteringAndDerivatives=provide  SimscapeFilterOrder=1  InputFilterTimeConstant=0.001  UdotUserProvided=0
  Solver Configuration1 : nesl_utility/Solver Configuration  PhysicalDomain=network_engine_domain  SubClassName=solver  LeftPortType=input  RightPortType=generic  Tones=[]  Harmonics=[]  SimulateNoise=off  Profile=off  UseLocalSampling=off  EnableSwitchedLinearOptims=on  FrequencyDomain=off  UseCCode=off  RelTol=0.001  AbsTol=0.001  MinStep=1e-09  ToWorkspace=off  RevertToSquareIcSolve=off  NumHomotopyIterations=100  PhasorMode=off  PhasorModeNumHarmonics=1  ConsistencySolver=NEWTON_XTOL_AFTER_FTOL  CanonicalOrdering=UNORDERED  OptimizeIntermediates=UNOPTIMIZED  IndexReductionMethod=DerivativeReplacement  DoDC=off  ResidualTolerance=1e-09  ConsistencyTolSource=GLOBAL  ConsistencyAbsTol=0.001  ConsistencyRelTol=0.001  ConsistencyTolFactor=1e-2  UseLocalSolver=on  LocalSolverChoice=NE_BACKWARD_EULER_ADVANCER  ResolveIndetEquations=on  FunctionEvalNumThread=1  LocalSolverSampleTime=1e-4  DoFixedCost=off  MaxNonlinIter=3  MaxModeIter=2  ComputeImpulses=off  ImpulseIterations=2  LinearAlgebra=auto  LinearAlgebraNumThread=0  EquationFormulation=NE_TIME_EF  DelaysMemoryBudget=1024  AutomaticFiltering=off  FilteringTimeConstant=0.001  PartitionStorageMethod=AS_NEEDED  PartitionMemoryBudget=1024  PartitionMethod=ROBUST  MultibodyUseLocalSolver=off  MultibodyLocalSolverChoice=ODE1  MultibodyLocalSolverSampleTime=0.001
  Terminator : Terminator
  Unit Delay{,1,3..4} (4 alike) : UnitDelay  SampleTime=-1
  Voltage Sensor : fl_lib/Electrical/Electrical Sensors/Voltage Sensor
  R : PMIOPort  Side=Left
  wires:
  Unit Delay4/1 -> PMSM Field-Oriented Control/2  "Current"
  [Current] -> Unit Delay4/1
  PS-Simulink Converter2/1 -> [Current]  "Current"
  [omga] -> Unit Delay/1
  [theta] -> Unit Delay1/1
  PS-Simulink Converter/1 -> [omga]  "rad/s"
  TorqueCommand/1 -> PMSM Field-Oriented Control/1  "Torque"
  PS-Simulink Converter1/1 -> [theta]  "rad"
  PS-Simulink Converter3/1 -> Unit Delay3/1
  PMSM Field-Oriented Control/1 -> Terminator/1
  Bus Selector/1 -> Simulink-PS Converter/1  "<modWave>"
  Unit Delay/1 -> PMSM Field-Oriented Control/3  "speed"
  Unit Delay1/1 -> PMSM Field-Oriented Control/4  "angle"
  Unit Delay3/1 -> PMSM Field-Oriented Control/5  "Vdc"
  PMSM Field-Oriented Control/2 -> Bus Selector/1
  connections:
  Average-Value Voltage Source Converter (Three-Phase)/RConn1 -- Voltage Sensor/LConn1 -- DC Voltage Source/LConn1
  Solver Configuration1/RConn1 -- Voltage Sensor/RConn2 -- Electrical Reference1/LConn1 -- Average-Value Voltage Source Converter (Three-Phase)/RConn2 -- DC Voltage Source/RConn1
  Current Sensor (Three-Phase)/LConn1 -- Average-Value Voltage Source Converter (Three-Phase)/LConn2
  Simulink-PS Converter/RConn1 -- Average-Value Voltage Source Converter (Three-Phase)/LConn1
  PS-Simulink Converter2/LConn1 -- Current Sensor (Three-Phase)/RConn1
  Voltage Sensor/RConn1 -- PS-Simulink Converter3/LConn1
  PMSM/LConn1 -- Current Sensor (Three-Phase)/RConn2
  Ideal Rotational Motion Sensor/RConn2 -- PS-Simulink Converter1/LConn1
  PMSM/RConn2 -- Mechanical Rotational Reference/LConn1
  Ideal Rotational Motion Sensor/LConn1 -- PMSM/RConn1 -- R/RConn1
  PS-Simulink Converter/LConn1 -- Ideal Rotational Motion Sensor/RConn1
